simulink model "INS"  (R2018b)
settings: configuration reference "ins_config" (kept outside this file)
values from neighbouring files (symbols this model uses):
  INS_EXPORT = Simulink.Parameter(INS_EXPORT_VALUE)    [ins_model_init.m]
  INS_PARAM = Simulink.Parameter(INS_PARAM_VALUE)    [ins_model_init.m]
undefined symbols (not defined in the file or in its folder): DiscIntNeverNeededParam, INS_CONST, INS_EXPORT_VALUE, Sensor_Meas
libraries: simulink x131, FMT_Model_Lib x48
(part 4 of 6)

== system INS/Data_Fusion/Translation_Filter/TF_Data_PreProcess/Sensor_Process/TF_Sensor_Status/ExternalPos_Status ==
  Sensor_Data : Inport
  Bus Creator : BusCreator  Inputs=2
  Bus Selector : BusSelector  OutputSignals=ExternalPos_Data.pos_valid,ExternalPos_Data.height_valid
  Signal Copy : SignalConversion  OverrideOpt=off
  Signal Copy1 : SignalConversion  OverrideOpt=off
  ExtPos_Status : Outport
  wires:
  Signal Copy/1 -> Bus Creator/1  "pos_valid"
  Sensor_Data/1 -> Bus Selector/1
  Bus Creator/1 -> ExtPos_Status/1
  Bus Selector/1 -> Signal Copy/1  "<pos_valid>"
  Bus Selector/2 -> Signal Copy1/1  "<height_valid>"
  Signal Copy1/1 -> Bus Creator/2  "height_valid"

== system INS/Data_Fusion/Translation_Filter/TF_Data_PreProcess/Sensor_Process/TF_Sensor_Status/GPS_Status ==
  Sensor_Data : Inport
  Rotation_Data : Inport  Port=2
  Bus Creator : BusCreator  Inputs=6
  Bus Selector : BusSelector  OutputSignals=GPS_Data.GPS_valid,GPS_Data.spd_quality,GPS_Data.pos_quality,GPS_Data.alt_quality,GPS_Data.fixType
  Bus Selector1 : BusSelector  OutputSignals=standstill
  Compare To Constant : simulink/Logic and Bit Operations/Compare To Constant  relop===  const=6  OutDataTypeStr=boolean
  Relay : Relay  OnSwitchValue=0.7  OffSwitchValue=0.4
  Relay1 : Relay  OnSwitchValue=0.7  OffSwitchValue=0.5
  Relay2 : Relay  OnSwitchValue=0.7  OffSwitchValue=0.6
  Signal Copy : SignalConversion  OverrideOpt=off
  Signal Copy1 : SignalConversion  OverrideOpt=off
  GPS_Status : Outport
  wires:
  Bus Creator/1 -> GPS_Status/1
  Relay1/1 -> Bus Creator/3  "pos_valid"
  Relay/1 -> Bus Creator/2  "spd_valid"
  Signal Copy/1 -> Bus Creator/1  "gps_vaid"
  Bus Selector/3 -> Relay1/1  "<pos_quality>"
  Bus Selector/2 -> Relay/1  "<spd_quality>"
  Bus Selector/1 -> Signal Copy/1  "<GPS_valid>"
  Sensor_Data/1 -> Bus Selector/1
  Bus Selector/4 -> Relay2/1  "<alt_quality>"
  Relay2/1 -> Bus Creator/4  "alt_valid"
  Bus Selector/5 -> Compare To Constant/1  "<fixType>"
  Compare To Constant/1 -> Bus Creator/5  "rtk_valid"
  Rotation_Data/1 -> Bus Selector1/1
  Bus Selector1/1 -> Signal Copy1/1  "<standstill>"
  Signal Copy1/1 -> Bus Creator/6  "standstill"

== system INS/Data_Fusion/Translation_Filter/TF_Data_PreProcess/Sensor_Process/TF_Sensor_Status/OpticalFlow_Status ==
  Sensor_Data : Inport
  Bus Creator : BusCreator  Inputs=1
  Bus Selector : BusSelector  OutputSignals=OpticalFlow_Data.valid
  Signal Copy : SignalConversion  OverrideOpt=off
  OptFlow_Status : Outport
  wires:
  Signal Copy/1 -> Bus Creator/1  "optflow_valid"
  Sensor_Data/1 -> Bus Selector/1
  Bus Creator/1 -> OptFlow_Status/1
  Bus Selector/1 -> Signal Copy/1  "<valid>"

== system INS/Data_Fusion/Translation_Filter/TF_Data_PreProcess/Sensor_Process/TF_Sensor_Status/Rangefinder_Status ==
  Sensor_Data : Inport
  Bus Creator : BusCreator  Inputs=1
  Bus Selector : BusSelector  OutputSignals=Rangefinder_Data.valid
  Signal Copy : SignalConversion  OverrideOpt=off
  Rf_Status : Outport
  wires:
  Bus Selector/1 -> Signal Copy/1  "<valid>"
  Bus Creator/1 -> Rf_Status/1
  Sensor_Data/1 -> Bus Selector/1
  Signal Copy/1 -> Bus Creator/1  "rf_valid"

== system INS/Data_Fusion/Translation_Filter/TF_Data_PreProcess/TF_Data_Post_Process/GPS_OFFSET_Compensation/GPS_POS_Compensation ==
  Rotation_Data : Inport
  TF_Data : Inport  Port=2
  GPS_Offset : Inport  Port=3
  Bus Selector1 : BusSelector  OutputSignals=M_OB
  Multiply2 : Product  Multiplication=Matrix(*)
  Reshape : Reshape  OutputDimensionality=Column vector (2-D)
  Sum1 : Sum  Inputs=|-+
  WGS_To_Global : Subsystem
  pos_O_m : Outport
  wires:
  WGS_To_Global/1(pos_O_m) -> Reshape/1
  TF_Data/1 -> WGS_To_Global/1(TF_Data)
  GPS_Offset/1 -> Multiply2/2
  Rotation_Data/1 -> Bus Selector1/1
  Bus Selector1/1 -> Multiply2/1  "<M_OB>"
  Reshape/1 -> Sum1/2
  Multiply2/1 -> Sum1/1
  Sum1/1 -> pos_O_m/1

== system INS/Data_Fusion/Translation_Filter/TF_Data_PreProcess/TF_Data_Post_Process/GPS_OFFSET_Compensation/GPS_VEL_Compensation ==
  Rotation_Data : Inport
  TF_Data : Inport  Port=2
  GPS_Offset : Inport  Port=3
  Bus Selector2 : BusSelector  OutputSignals=M_OB
  Bus Selector3 : BusSelector  OutputSignals=Sensor_Meas.GPS_Meas.vn_mPs,Sensor_Meas.GPS_Meas.ve_mPs,Sensor_Meas.GPS_Meas.vd_mPs
  Bus Selector4 : BusSelector  OutputSignals=gyr_B_radPs
  Cross Product : FMT_Model_Lib/Math/Cross Product
      settings: SourceProductName=FMT Toolbox
  Multiply4 : Product  Multiplication=Matrix(*)
  Mux1 : Mux  Inputs=3
  Reshape : Reshape  OutputDimensionality=Column vector (2-D)
  Sum : Sum  Inputs=+-|
  delay : Subsystem
  vel_O_mPs : Outport
  wires:
  Bus Selector3/3 -> Mux1/3  "<vd_mPs>"
  Bus Selector3/2 -> Mux1/2  "<ve_mPs>"
  Mux1/1 -> Reshape/1
  TF_Data/1 -> Bus Selector3/1
  Rotation_Data/1 -> Bus Selector2/1, Bus Selector4/1
  Bus Selector4/1 -> Cross Product/1  "<gyr_B_radPs>"
  Bus Selector3/1 -> Mux1/1  "<vn_mPs>"
  GPS_Offset/1 -> Cross Product/2
  Reshape/1 -> Sum/1
  Bus Selector2/1 -> Multiply4/1  "<M_OB>"
  Multiply4/1 -> Sum/2
  Cross Product/1 -> delay/1(u)  "gps_vel_offset"
  delay/1(y) -> Multiply4/2
  Sum/1 -> vel_O_mPs/1

== system INS/Data_Fusion/Translation_Filter/TF_Data_PreProcess/Transfer_Filter_Control/Sensor_Valid/Horizon_Sensor_Valid ==
  Sensor_Enable : Inport
  Bus Selector1 : BusSelector  OutputSignals=horizon_select.gps_enable,horizon_select.optflow_enable,horizon_select.extpos_enable,horizon_select.airspeed_enable
  Logical Operator : Logic  Operator=OR  Inputs=3  AllPortsSameDT=off  OutDataTypeStr=boolean
  valid_hold : Subsystem  mask{time_out=1000}
      mask prompts: time_out "timeout in ms"
  valid_hold1 : Subsystem  mask{time_out=1000}
      mask prompts: time_out "timeout in ms"
  valid_hold2 : Subsystem  mask{time_out=1000}
      mask prompts: time_out "timeout in ms"
  lon_lat_valid : Outport
  xy_R_valid : Outport  Port=2
  airspeed_valid : Outport  Port=3
  wires:
  Sensor_Enable/1 -> Bus Selector1/1
  Bus Selector1/1 -> Logical Operator/1, valid_hold/1(u)  "<gps_enable>"
  valid_hold/1(y) -> lon_lat_valid/1
  valid_hold1/1(y) -> xy_R_valid/1
  Bus Selector1/2 -> Logical Operator/2  "<optflow_enable>"
  Logical Operator/1 -> valid_hold1/1(u)
  Bus Selector1/3 -> Logical Operator/3  "<extpos_enable>"
  valid_hold2/1(y) -> airspeed_valid/1
  Bus Selector1/4 -> valid_hold2/1(u)  "<airspeed_enable>"

== system INS/Data_Fusion/Translation_Filter/TF_Data_PreProcess/Transfer_Filter_Control/Sensor_Valid/Vertical_Sensor_Valid ==
  Sensor_Enable : Inport
  Bus Selector1 : BusSelector  OutputSignals=vert_select.gps_enable,vert_select.baro_enable,vert_select.extpos_enable,vert_select.rf_enable
  Logical Operator : Logic  Operator=OR  Inputs=4  AllPortsSameDT=off  OutDataTypeStr=boolean
  valid_hold : Subsystem  mask{time_out=1000}
      mask prompts: time_out "timeout in ms"
  valid_hold1 : Subsystem  mask{time_out=1000}
      mask prompts: time_out "timeout in ms"
  valid_hold2 : Subsystem  mask{time_out=1000}
      mask prompts: time_out "timeout in ms"
  altitude_valid : Outport
  h_R_valid : Outport  Port=2
  h_AGL_valid : Outport  Port=3
  wires:
  Sensor_Enable/1 -> Bus Selector1/1
  Bus Selector1/1 -> Logical Operator/1, valid_hold/1(u)  "<gps_enable>"
  Bus Selector1/2 -> Logical Operator/2  "<baro_enable>"
  Logical Operator/1 -> valid_hold1/1(u)
  valid_hold/1(y) -> altitude_valid/1
  valid_hold1/1(y) -> h_R_valid/1
  Bus Selector1/4 -> Logical Operator/4, valid_hold2/1(u)  "<rf_enable>"
  valid_hold2/1(y) -> h_AGL_valid/1
  Bus Selector1/3 -> Logical Operator/3  "<extpos_enable>"

== system INS/Data_Fusion/Translation_Filter/TF_Data_PreProcess/Transfer_Filter_Control/WGS84_Reference/Bus_Constructor ==
  WGS84_pos_ref : Inport
  WGS84_dpos_ref : Inport  Port=2
  WGS84_hgt_ref : Inport  Port=3
  WGS84_dhgt_ref : Inport  Port=4
  Bus Creator : BusCreator  Inputs=2
  Bus Creator1 : BusCreator  Inputs=3
  Bus Creator2 : BusCreator  Inputs=3
  Demux : Demux  Outputs=2
  Demux1 : Demux  Outputs=2
  WGS84_Ref : Outport
  wires:
  Bus Creator/1 -> WGS84_Ref/1
  Demux/1 -> Bus Creator1/1  "dx_dlat_0"
  Demux1/1 -> Bus Creator2/1  "lat_0_rad"
  Demux/2 -> Bus Creator1/2  "dy_dlon_0"
  Demux1/2 -> Bus Creator2/2  "lon_0_rad"
  Bus Creator2/1 -> Bus Creator/2  "WGS84_pos_ref"
  WGS84_dhgt_ref/1 -> Bus Creator1/3  "dz_dh_0"
  WGS84_hgt_ref/1 -> Bus Creator2/3  "h_0_m"
  Bus Creator1/1 -> Bus Creator/1  "WGS84_derivatives_ref"
  WGS84_dpos_ref/1 -> Demux/1
  WGS84_pos_ref/1 -> Demux1/1

== system INS/Data_Fusion/Translation_Filter/TF_Data_PreProcess/Transfer_Filter_Control/WGS84_Reference/Bus_Select ==
  Sensor_Meas : Inport
  Bus Selector1 : BusSelector  OutputSignals=GPS_Meas.dx_dlat,GPS_Meas.dy_dlon,GPS_Meas.dz_dh,GPS_Meas.lat_rad,GPS_Meas.lon_rad,GPS_Meas.h_m
  Mux : Mux  Inputs=3
  Mux1 : Mux  Inputs=3
  WGS84_derivatives : Outport
  WGS84_position : Outport  Port=2
  wires:
  Mux1/1 -> WGS84_position/1
  Sensor_Meas/1 -> Bus Selector1/1
  Mux/1 -> WGS84_derivatives/1
  Bus Selector1/6 -> Mux1/3  "<h_m>"
  Bus Selector1/5 -> Mux1/2  "<lon_rad>"
  Bus Selector1/4 -> Mux1/1  "<lat_rad>"
  Bus Selector1/3 -> Mux/3  "<dz_dh>"
  Bus Selector1/2 -> Mux/2  "<dy_dlon>"
  Bus Selector1/1 -> Mux/1  "<dx_dlat>"

== system INS/Data_Fusion/Translation_Filter/TF_Data_PreProcess/Transfer_Filter_Control/WGS84_Reference/Height_Ref ==
  Translation_Data : Inport
  Sensor_Valid : Inport  Port=2
  WGS84_derivatives : Inport  Port=3
  WGS84_position : Inport  Port=4
  Bus Selector1 : BusSelector  OutputSignals=h_R_m
  Bus Selector2 : BusSelector  OutputSignals=altitude_valid
  Delay : Delay  DelayLength=1
  Delay1 : Delay  DelayLength=1
  Detect Rise Positive3 : simulink/Logic and Bit Operations/Detect Rise Positive  vinit=0  OutDataTypeStr=boolean
  Selector : Selector  InputPortWidth=3  IndexOptions=Index vector (dialog)  Indices=3  OutputSizes=1
  Selector1 : Selector  InputPortWidth=3  IndexOptions=Index vector (dialog)  Indices=3  OutputSizes=1
  Sum : Sum  Inputs=|+-
  Switch1 : Switch  Criteria=u2 > Threshold
  Switch4 : Switch  Criteria=u2 > Threshold
  WGS84_hgt_ref : Outport
  WGS84_dhgt_ref : Outport  Port=2
  wires:
  Delay1/1 -> Switch4/3
  Switch4/1 -> WGS84_hgt_ref/1, Delay1/1
  Detect Rise Positive3/1 -> Switch1/2, Switch4/2
  Bus Selector2/1 -> Detect Rise Positive3/1  "<altitude_valid>"
  WGS84_derivatives/1 -> Selector/1
  Switch1/1 -> WGS84_dhgt_ref/1, Delay/1
  Delay/1 -> Switch1/3
  Sensor_Valid/1 -> Bus Selector2/1
  Translation_Data/1 -> Bus Selector1/1
  Sum/1 -> Switch4/1
  WGS84_position/1 -> Selector1/1
  Selector/1 -> Switch1/1
  Selector1/1 -> Sum/1
  Bus Selector1/1 -> Sum/2  "<h_R_m>"

== system INS/Data_Fusion/Translation_Filter/TF_Data_PreProcess/Transfer_Filter_Control/WGS84_Reference/Position_Ref ==
  Translation_Data : Inport
  Sensor_Valid : Inport  Port=2
  WGS84_derivatives : Inport  Port=3
  WGS84_position : Inport  Port=4
  Bus Selector1 : BusSelector  OutputSignals=x_R_m,y_R_m
  Bus Selector2 : BusSelector  OutputSignals=lon_lat_valid
  Delay : Delay  DelayLength=1
  Delay1 : Delay  DelayLength=1
  Detect Rise Positive3 : simulink/Logic and Bit Operations/Detect Rise Positive  vinit=0  OutDataTypeStr=boolean
  Divide : Product  Inputs=*/
  Mux : Mux  Inputs=2
  Selector : Selector  InputPortWidth=3  IndexOptions=Index vector (dialog)  Indices=[1 2]  OutputSizes=1
  Selector1 : Selector  InputPortWidth=3  IndexOptions=Index vector (dialog)  Indices=[1 2]  OutputSizes=1
  Sum : Sum  Inputs=|+-
  Switch1 : Switch  Criteria=u2 > Threshold
  Switch4 : Switch  Criteria=u2 > Threshold
  WGS84_pos_ref : Outport
  WGS84_dpos_ref : Outport  Port=2
  wires:
  Delay/1 -> Switch4/3
  Bus Selector1/1 -> Mux/1  "<x_R_m>"
  Switch4/1 -> WGS84_pos_ref/1, Delay/1
  Mux/1 -> Divide/1  "dxdy"
  Detect Rise Positive3/1 -> Switch1/2, Switch4/2
  Bus Selector2/1 -> Detect Rise Positive3/1  "<lon_lat_valid>"
  WGS84_derivatives/1 -> Selector/1
  Switch1/1 -> Delay1/1, WGS84_dpos_ref/1
  Delay1/1 -> Switch1/3
  Sensor_Valid/1 -> Bus Selector2/1
  Translation_Data/1 -> Bus Selector1/1
  Sum/1 -> Switch4/1
  Bus Selector1/2 -> Mux/2  "<y_R_m>"
  Divide/1 -> Sum/2  "dlat_dlon"
  WGS84_position/1 -> Selector1/1
  Selector/1 -> Switch1/1, Divide/2  "dxdy_dlatdlon"
  Selector1/1 -> Sum/1

== system INS/Sensor_PreProcess/MAG_PreProcess/Mag_Data_Process/Mag_Quality_Estimate/Mag_Quality/Inclination_Quality_Estimate ==
  nominal_inc_deg : Inport
  mag_normalized_O : Inport  Port=2
  Abs1 : Abs
  Constant2 : Constant  OutDataTypeStr=Inherit: Inherit via back propagation
  Gain1 : Gain  Gain=pi/180
  Saturation : Saturate  UpperLimit=1  LowerLimit=0
  Selector : Selector  InputPortWidth=3  IndexOptions=Index vector (dialog)  Indices=[1 2]  OutputSizes=1
  Selector1 : Selector  InputPortWidth=3  IndexOptions=Index vector (dialog)  Indices=3  OutputSizes=1
  Subtract : Sum  Inputs=+-
  Sum3 : Sum  Inputs=+-|
  Trigonometric Function : Trigonometry  Operator=atan2
  Vector Modulus : FMT_Model_Lib/Math/Vector Modulus
      settings: SourceProductName=FMT Toolbox
  gain : Gain  Gain=2
  inclination_quality : Outport
  wires:
  mag_normalized_O/1 -> Selector1/1, Selector/1
  Trigonometric Function/1 -> Subtract/2
  Vector Modulus/1 -> Trigonometric Function/2
  Abs1/1 -> gain/1
  gain/1 -> Sum3/2
  Gain1/1 -> Subtract/1
  Subtract/1 -> Abs1/1
  Constant2/1 -> Sum3/1
  nominal_inc_deg/1 -> Gain1/1
  Sum3/1 -> Saturation/1
  Selector/1 -> Vector Modulus/1
  Selector1/1 -> Trigonometric Function/1
  Saturation/1 -> inclination_quality/1

== system INS/Sensor_PreProcess/MAG_PreProcess/Mag_Data_Process/Mag_Quality_Estimate/Mag_Quality/Intensity_Quality_Estimate ==
  mag_normalized_O : Inport
  Abs : Abs
  Constant1 : Constant  OutDataTypeStr=Inherit: Inherit via back propagation
  Nominal_Magnitude : Constant  OutDataTypeStr=Inherit: Inherit via back propagation
  Saturation : Saturate  UpperLimit=1  LowerLimit=0
  Subtract : Sum  Inputs=+-
  Sum : Sum  Inputs=+-|
  Vector Modulus : FMT_Model_Lib/Math/Vector Modulus
      settings: SourceProductName=FMT Toolbox
  gain : Gain
  intensity_quality : Outport
  wires:
  Constant1/1 -> Sum/1
  Vector Modulus/1 -> Subtract/2
  Subtract/1 -> Abs/1
  Sum/1 -> Saturation/1
  Nominal_Magnitude/1 -> Subtract/1
  Saturation/1 -> intensity_quality/1
  Abs/1 -> gain/1  "magnitude_error"
  gain/1 -> Sum/2
  mag_normalized_O/1 -> Vector Modulus/1

== system INS/Data_Fusion/Rotation_Filter/AHRS/Correct/Attitude_Correction/Attitude_Correct/Acc_Correct ==
  acc_meas_valid : Inport
  acc_meas_O_mPs2 : Inport  Port=2
  acc_est_O_mPs2 : Inport  Port=3
  Heading_Correct : Subsystem
  Sum : Sum  Inputs=|++
  Verticle_Correct : Subsystem
  att_correct : Outport
  wires:
  acc_meas_valid/1 -> Heading_Correct/3(acc_meas_valid)
  Verticle_Correct/1(vert_correct) -> Sum/1  "vert_correct"
  Heading_Correct/1(heading_correct) -> Sum/2  "heading_correct"
  acc_meas_O_mPs2/1 -> Verticle_Correct/2(acc_meas_O_mPs2), Heading_Correct/2(acc_meas_O_mPs2)
  acc_est_O_mPs2/1 -> Verticle_Correct/1(acc_est_O_mPs2), Heading_Correct/1(acc_est_O_mPs2)
  Sum/1 -> att_correct/1

== system INS/Data_Fusion/Rotation_Filter/AHRS/Correct/Attitude_Correction/Attitude_Correct/Acc_Estimator ==
  RF_Data : Inport
  Sensor_Data : Inport  Port=2
  Rotation_Data : Inport  Port=3
  Estimate_Acc : Subsystem
  Measure_Acc : Subsystem
  Multiply : Product  OutDataTypeStr=single
  Sum2 : Sum  Inputs=++|
  gravity : Constant  Value=[0;0;-INS_CONST.g]  VectorParams1D=off  OutDataTypeStr=single
  acc_meas_valid : Outport
  acc_meas_O_mPs2 : Outport  Port=2
  acc_est_O_mPs2 : Outport  Port=3
  wires:
  Measure_Acc/1(gps_meas_valid) -> Estimate_Acc/1(gps_meas_valid), acc_meas_valid/1, Multiply/1
  Sum2/1 -> acc_meas_O_mPs2/1
  Sensor_Data/1 -> Estimate_Acc/2(Sensor_Data), Measure_Acc/2(Sensor_Data)
  gravity/1 -> Sum2/1
  Multiply/1 -> Sum2/2
  Measure_Acc/2(gps_meas_acc) -> Multiply/2
  Rotation_Data/1 -> Estimate_Acc/3(Rotation_Data)
  Estimate_Acc/1(acc_est_O_mPs2) -> acc_est_O_mPs2/1
  RF_Data/1 -> Measure_Acc/1(RF_Data)

== system INS/Data_Fusion/Rotation_Filter/AHRS/Correct/Attitude_Correction/ExternalPsi_Correct/Bias_Estimation ==
  bias_update : Inport
  psi_meas : Inport  Port=2
  psi_est : Inport  Port=3
  Bias : Subsystem
  Constant : Constant  Value=INS_PARAM.EXT_PSI_BIAS_EST_EN
  Delay : Delay  DelayLength=1
  Multiply : Product
  Switch : Switch  Criteria=u2 > Threshold  OutDataTypeStr=single
  bias : Outport
  wires:
  Delay/1 -> Switch/3
  Bias/1(bias) -> Switch/1
  Multiply/1 -> Delay/1, bias/1
  psi_meas/1 -> Bias/2(psi_meas)
  psi_est/1 -> Bias/1(psi_est)
  bias_update/1 -> Switch/2  "ext_psi_bias_update"
  Switch/1 -> Multiply/2
  Constant/1 -> Multiply/1

== system INS/Data_Fusion/Rotation_Filter/AHRS/Correct/Attitude_Correction/ExternalPsi_Correct/psi_err_saturation ==
  psi_err_in : Inport
  Abs : Abs
  Compare To Constant : simulink/Logic and Bit Operations/Compare To Constant  relop=>  const=pi  OutDataTypeStr=boolean
  Constant : Constant  Value=2*pi  OutDataTypeStr=single
  Multiply : Product
  Sign : Signum
  Subtract : Sum  Inputs=-+
  Switch : Switch  Criteria=u2 > Threshold
  psi_err_rad : Outport
  wires:
  Multiply/1 -> Switch/1
  Sign/1 -> Multiply/2
  Subtract/1 -> Multiply/1
  Constant/1 -> Subtract/1
  Switch/1 -> psi_err_rad/1
  Compare To Constant/1 -> Switch/2
  Abs/1 -> Compare To Constant/1, Subtract/2
  psi_err_in/1 -> Abs/1, Switch/3, Sign/1

== system INS/Data_Fusion/Rotation_Filter/AHRS/Correct/Attitude_Correction/GPS_Heading_Correct/psi_err_saturation ==
  psi_err_in : Inport
  Abs : Abs
  Compare To Constant : simulink/Logic and Bit Operations/Compare To Constant  relop=>  const=pi  OutDataTypeStr=boolean
  Constant : Constant  Value=2*pi  OutDataTypeStr=single
  Multiply : Product
  Sign : Signum
  Subtract : Sum  Inputs=-+
  Switch : Switch  Criteria=u2 > Threshold
  psi_err_rad : Outport
  wires:
  Multiply/1 -> Switch/1
  Sign/1 -> Multiply/2
  Subtract/1 -> Multiply/1
  Constant/1 -> Subtract/1
  Switch/1 -> psi_err_rad/1
  Compare To Constant/1 -> Switch/2
  Abs/1 -> Compare To Constant/1, Subtract/2
  psi_err_in/1 -> Abs/1, Switch/3, Sign/1

== system INS/Data_Fusion/Rotation_Filter/AHRS/Correct/Attitude_Correction/Mag_Correct/Mag_Control ==
  RF_Data : Inport
  Rotation_Data : Inport  Port=2
  Sensor_Data : Inport  Port=3
  Translation_Data : Inport  Port=4
  Bus Selector3 : BusSelector  OutputSignals=mag_enable
  Detect Increase1 : simulink/Logic and Bit Operations/Detect Increase  vinit=0.0  OutDataTypeStr=boolean
  Hover : Subsystem
  Hover_Mag_Correcrt : Subsystem
  Logical Operator4 : Logic  Operator=OR  AllPortsSameDT=off  OutDataTypeStr=boolean
  use_mag : Outport
  mag_bias_update : Outport  Port=2
  wires:
  Rotation_Data/1 -> Hover/1(Rotation_Data)
  Detect Increase1/1 -> mag_bias_update/1  "mag_bias_update"
  RF_Data/1 -> Hover_Mag_Correcrt/1(RF_Data), Bus Selector3/1
  Bus Selector3/1 -> Logical Operator4/1  "<mag_enable>"
  Logical Operator4/1 -> Detect Increase1/1, use_mag/1  "use_mag"
  Translation_Data/1 -> Hover/2(Translation_Data)
  Sensor_Data/1 -> Hover_Mag_Correcrt/2(Sensor_Data)
  Hover/1(hover) -> Hover_Mag_Correcrt/3(hover)  "hover"
  Hover_Mag_Correcrt/1(use_mag_when_hover) -> Logical Operator4/2

== system INS/Data_Fusion/Rotation_Filter/AHRS/Correct/Attitude_Correction/Mag_Correct/Mag_Measure ==
  bias_update : Inport
  mag_norm_B : Inport  Port=2
  Rotation_Data : Inport  Port=3
  Bias_Estimation : Subsystem
  Bus Selector : BusSelector  OutputSignals=psi_rad,standstill
  Mag_Heading : Subsystem
  Sum : Sum  Inputs=++|
  psi_meas : Outport
  wires:
  Mag_Heading/1(mag_psi) -> Sum/1, Bias_Estimation/2(psi_meas)
  Rotation_Data/1 -> Mag_Heading/2(Rotation_Data), Bus Selector/1
  mag_norm_B/1 -> Mag_Heading/1(mag_B)
  Bus Selector/1 -> Bias_Estimation/3(psi_est)  "<psi_rad>"
  Sum/1 -> psi_meas/1
  Bias_Estimation/1(bias) -> Sum/2  "psi_bias"
  bias_update/1 -> Bias_Estimation/1(bias_update)
  Bus Selector/2 -> Bias_Estimation/4(standstill)  "<standstill>"

== system INS/Data_Fusion/Rotation_Filter/AHRS/Correct/Attitude_Correction/Mag_Correct/psi_err_saturation ==
  psi_err_in : Inport
  Abs : Abs
  Compare To Constant : simulink/Logic and Bit Operations/Compare To Constant  relop=>  const=pi  OutDataTypeStr=boolean
  Constant : Constant  Value=2*pi  OutDataTypeStr=single
  Multiply : Product
  Sign : Signum
  Subtract : Sum  Inputs=-+
  Switch : Switch  Criteria=u2 > Threshold
  psi_err_rad : Outport
  wires:
  Multiply/1 -> Switch/1
  Sign/1 -> Multiply/2
  Subtract/1 -> Multiply/1
  Constant/1 -> Subtract/1
  Switch/1 -> psi_err_rad/1
  Compare To Constant/1 -> Switch/2
  Abs/1 -> Compare To Constant/1, Subtract/2
  psi_err_in/1 -> Abs/1, Switch/3, Sign/1

== system INS/Data_Fusion/Translation_Filter/CF/Bus_Constructor/Bus_Select/WGS84_Position/WGS84_Position ==
  xyh_R_m : Inport
  TF_Data : Inport  Port=2
  Bus Selector : BusSelector  OutputSignals=TF_Control.WGS84_Ref.WGS84_derivatives_ref.dx_dlat_0,TF_Control.WGS84_Ref.WGS84_derivatives_ref.dy_dlon_0
  Bus Selector1 : BusSelector  OutputSignals=TF_Control.WGS84_Ref.WGS84_pos_ref.lat_0_rad,TF_Control.WGS84_Ref.WGS84_pos_ref.lon_0_rad,TF_Control.WGS84_Ref.WGS84_pos_ref.h_0_m
  Data Type Conversion : DataTypeConversion  OutDataTypeStr=double
  Data Type Conversion1 : DataTypeConversion  OutDataTypeStr=double
  Mux : Mux  Inputs=2
  Mux1 : Mux  Inputs=2
  Mux2 : Mux  Inputs=3
  Selector : Selector  InputPortWidth=3  IndexOptions=Index vector (dialog)  Indices=[1 2]  OutputSizes=1
  Selector1 : Selector  InputPortWidth=3  IndexOptions=Index vector (dialog)  Indices=[3]  OutputSizes=1
  Sum : Sum  Inputs=|++
  safe_divide : Subsystem
  WGS84_pos : Outport
  wires:
  Selector/1 -> Data Type Conversion/1
  Mux/1 -> safe_divide/2(u2)
  Selector1/1 -> Data Type Conversion1/1
  Data Type Conversion1/1 -> Mux1/2
  Bus Selector/1 -> Mux/1  "<dx_dlat_0>"
  xyh_R_m/1 -> Selector1/1, Selector/1
  Bus Selector/2 -> Mux/2  "<dy_dlon_0>"
  safe_divide/1(y) -> Mux1/1
  Data Type Conversion/1 -> safe_divide/1(u1)
  Mux1/1 -> Sum/1
  Bus Selector1/2 -> Mux2/2  "<lon_0_rad>"
  TF_Data/1 -> Bus Selector1/1, Bus Selector/1
  Bus Selector1/3 -> Mux2/3  "<h_0_m>"
  Bus Selector1/1 -> Mux2/1  "<lat_0_rad>"
  Mux2/1 -> Sum/2
  Sum/1 -> WGS84_pos/1

== system INS/Data_Fusion/Translation_Filter/CF/Horizontal_Filter/Correct/Airspeed Correct/Airspeed_Correct ==
  TF_Data : Inport
  X_Predict : Inport  Port=2
  Enable : EnablePort  StatesWhenEnabling=reset
  Bus Selector : BusSelector  OutputSignals=TF_Control.sensor_valid.airspeed_valid
  Bus Selector1 : BusSelector  OutputSignals=Sensor_Meas.Airspeed_Meas.timestamp_ms
  Detect Change : simulink/Logic and Bit Operations/Detect Change  vinit=0  OutDataTypeStr=boolean
  Detect Increase : simulink/Logic and Bit Operations/Detect Increase  vinit=0.0  OutDataTypeStr=boolean
  Error_Integrate : Subsystem
  Error_Scaling : Subsystem
  Estimate_State : Subsystem
  Measurement : Subsystem
  Sum : Sum  Inputs=|-+
  Sum1 : Sum  Inputs=++|
  X_Next : Outport
  wires:
  Error_Scaling/1(err_out) -> Error_Integrate/1(error)
  Detect Change/1 -> Error_Integrate/2(update)
  Bus Selector/1 -> Detect Increase/1  "<airspeed_valid>"
  X_Predict/1 -> Sum1/1, Estimate_State/1(X)
  Sum1/1 -> X_Next/1
  Error_Integrate/1(corr) -> Sum1/2
  Bus Selector1/1 -> Detect Change/1  "<timestamp_ms>"
  Sum/1 -> Error_Scaling/1(err_in)  "airspeed_error_hor_O"
  TF_Data/1 -> Bus Selector1/1, Bus Selector/1, Measurement/1(TF_Data)
  Measurement/1(Z) -> Sum/2  "airspeed_meas_hor_O"
  Estimate_State/1(HX) -> Sum/1  "airspeed_state_hor_O"
  Detect Increase/1 -> Estimate_State/2(reset)

== system INS/Data_Fusion/Translation_Filter/CF/Horizontal_Filter/Correct/ExternalPos Correct/ExternalPos_Correct ==
  TF_Data : Inport
  X_Predict : Inport  Port=2
  Enable : EnablePort  StatesWhenEnabling=reset
  Bus Selector : BusSelector  OutputSignals=TF_Control.pos_reset
  Bus Selector1 : BusSelector  OutputSignals=Sensor_Meas.ExtPos_Meas.timestamp_ms
  Detect Change : simulink/Logic and Bit Operations/Detect Change  vinit=0  OutDataTypeStr=boolean
  Error_Integrate : Subsystem
  Error_Scaling : Subsystem
  Estimate_State : Subsystem
  Logical Operator : Logic  Operator=OR  AllPortsSameDT=off  OutDataTypeStr=boolean
  Measurement : Subsystem
  Sum : Sum  Inputs=|-+
  Sum1 : Sum  Inputs=++|
  X_Next : Outport
  wires:
  Estimate_State/1(HX) -> Sum/1  "extpos_state_hor_O"
  Measurement/1(Z) -> Sum/2  "extpos_meas_hor_O"
  TF_Data/1 -> Measurement/2(TF_Data), Bus Selector/1, Bus Selector1/1
  Sum/1 -> Error_Scaling/1(err_in)  "extpos_error_hor_O"
  Bus Selector1/1 -> Detect Change/1  "<timestamp_ms>"
  Error_Integrate/1(corr) -> Sum1/2  "corr_1"
  Sum1/1 -> X_Next/1
  X_Predict/1 -> Measurement/1(X), Estimate_State/1(X), Sum1/1
  Bus Selector/1 -> Estimate_State/2(reset)  "<pos_reset>"
  Logical Operator/1 -> Error_Integrate/2(update)
  Detect Change/1 -> Logical Operator/2
  Measurement/2(bias_update) -> Logical Operator/1
  Error_Scaling/1(err_out) -> Error_Integrate/1(error)

== system INS/Data_Fusion/Translation_Filter/CF/Horizontal_Filter/Correct/GPS Correct/GPS_Correct ==
  TF_Data : Inport
  X_Predict : Inport  Port=2
  Enable : EnablePort  StatesWhenEnabling=reset
  Bus Selector : BusSelector  OutputSignals=TF_Control.pos_reset
  Bus Selector1 : BusSelector  OutputSignals=Sensor_Meas.GPS_Meas.timestamp_ms
  Bus Selector2 : BusSelector  OutputSignals=Sensor_Status.GPS_Status.rtk_valid
  Detect Change : simulink/Logic and Bit Operations/Detect Change  vinit=0  OutDataTypeStr=boolean
  Error_Integrate : Subsystem
  Error_Scaling : Subsystem
  Estimate_State : Subsystem
  Logical Operator : Logic  Operator=OR  AllPortsSameDT=off  OutDataTypeStr=boolean
  Measurement : Subsystem
  Sum : Sum  Inputs=|-+
  Sum1 : Sum  Inputs=++|
  X_Next : Outport
  wires:
  Estimate_State/1(HX) -> Sum/1  "gps_state_hor_O"
  Measurement/1(Z) -> Sum/2  "gps_meas_hor_O"
  TF_Data/1 -> Bus Selector2/1, Bus Selector/1, Measurement/2(TF_Data), Bus Selector1/1
  Sum/1 -> Error_Scaling/1(err_in)  "gps_error_hor_O"
  Bus Selector1/1 -> Detect Change/1  "<timestamp_ms>"
  Error_Integrate/1(corr) -> Sum1/2
  Sum1/1 -> X_Next/1
  X_Predict/1 -> Estimate_State/1(X), Measurement/1(X), Sum1/1
  Bus Selector/1 -> Estimate_State/2(reset)  "<pos_reset>"
  Logical Operator/1 -> Error_Integrate/2(update)
  Detect Change/1 -> Logical Operator/2
  Measurement/2(bias_update) -> Logical Operator/1
  Error_Scaling/1(err_out) -> Error_Integrate/1(error)
  Bus Selector2/1 -> Error_Scaling/2(rtk_valid)  "<rtk_valid>"

== system INS/Data_Fusion/Translation_Filter/CF/Horizontal_Filter/Correct/OptFlow Correct/OptFlow_Correct ==
  TF_Data : Inport
  X_Predict : Inport  Port=2
  Enable : EnablePort  StatesWhenEnabling=reset
  Bus Selector : BusSelector  OutputSignals=TF_Control.pos_reset
  Bus Selector1 : BusSelector  OutputSignals=Sensor_Meas.OptFlow_Meas.timestamp_ms
  Detect Change : simulink/Logic and Bit Operations/Detect Change  vinit=0  OutDataTypeStr=boolean
  Error_Integrate : Subsystem
  Error_Scaling : Subsystem
  Estimate_State : Subsystem
  Measurement : Subsystem
  Sum : Sum  Inputs=|-+
  Sum1 : Sum  Inputs=++|
  X_Next : Outport
  wires:
  Estimate_State/1(HX) -> Sum/1  "optflow_state_O"
  Measurement/1(Z) -> Sum/2  "optflow_meas_O"
  TF_Data/1 -> Bus Selector1/1, Bus Selector/1, Measurement/1(TF_Data)
  Sum/1 -> Error_Scaling/1(err_in)  "optflow_error_O"
  Bus Selector1/1 -> Detect Change/1  "<timestamp_ms>"
  Error_Integrate/1(corr) -> Sum1/2
  Sum1/1 -> X_Next/1
  X_Predict/1 -> Estimate_State/1(X), Sum1/1
  Bus Selector/1 -> Estimate_State/2(reset)  "<pos_reset>"
  Detect Change/1 -> Error_Integrate/2(update)
  Error_Scaling/1(err_out) -> Error_Integrate/1(error)

== system INS/Data_Fusion/Translation_Filter/CF/Horizontal_Filter/Predict/Propagate/States_Init ==
  TF_Data : Inport
  Constant : Constant  Value=[0;0]  VectorParams1D=off  OutDataTypeStr=single
  Constant1 : Constant  Value=0  VectorParams1D=off  OutDataTypeStr=single
  Mux : Mux
  Pos_Init : Subsystem
  Vel_Init : Subsystem
  X_0 : Outport
  wires:
  TF_Data/1 -> Pos_Init/1(TF_Data), Vel_Init/1(TF_Data)
  Constant/1 -> Mux/3  "ba_xy_0"
  Mux/1 -> X_0/1
  Vel_Init/1(vel_NE_0) -> Mux/2  "vel_ne_0"
  Pos_Init/1(XY_0) -> Mux/1  "pos_xy_0"
  Constant1/1 -> Mux/4  "TAS"

== system INS/Data_Fusion/Translation_Filter/CF/Verticle_Filter/Correct/Baro_Correct/Baro_Correct ==
  TF_Data : Inport
  X_Predict : Inport  Port=2
  Enable : EnablePort  StatesWhenEnabling=reset
  Bus Selector : BusSelector  OutputSignals=TF_Control.height_reset
  Bus Selector1 : BusSelector  OutputSignals=Sensor_Meas.Baro_Meas.timestamp_ms
  Demux : Demux  Outputs=3
  Detect Change : simulink/Logic and Bit Operations/Detect Change  vinit=0  OutDataTypeStr=boolean
  Error_Hold : Subsystem
  Error_Scaling : Subsystem  mask{w=1.2}
      mask prompts: w "omega"
  Estimate_States : Subsystem
  Logical Operator : Logic  Operator=OR  AllPortsSameDT=off  OutDataTypeStr=boolean
  Measurement : Subsystem
  Mux : Mux  Inputs=3
  Saturation : Saturate
  Sum : Sum  Inputs=|-+
  Sum1 : Sum  Inputs=++|
  X_Next : Outport
  wires:
  Estimate_States/1(HX) -> Sum/1  "baro_state_vert_O"
  Measurement/1(Z) -> Sum/2  "baro_meas_vert_O"
  TF_Data/1 -> Bus Selector/1, Measurement/2(TF_Data), Bus Selector1/1
  Sum/1 -> Error_Scaling/1(errror_in)  "baro_error_vert_O"
  Bus Selector1/1 -> Detect Change/1  "<timestamp_ms>"
  Error_Hold/1(out) -> Sum1/2
  Sum1/1 -> Demux/1
  X_Predict/1 -> Measurement/1(X), Estimate_States/1(X), Sum1/1
  Bus Selector/1 -> Estimate_States/2(reset)  "<height_reset>"
  Logical Operator/1 -> Error_Hold/2(update)
  Detect Change/1 -> Logical Operator/2
  Measurement/2(bias_update) -> Logical Operator/1
  Error_Scaling/1(errror_out) -> Error_Hold/1(in)
  Demux/3 -> Saturation/1
  Mux/1 -> X_Next/1
  Saturation/1 -> Mux/3
  Demux/2 -> Mux/2
  Demux/1 -> Mux/1

== system INS/Data_Fusion/Translation_Filter/CF/Verticle_Filter/Correct/ExternalPos_Correct/ExternalPos_Correct ==
  TF_Data : Inport
  X_Predict : Inport  Port=2
  Enable : EnablePort  StatesWhenEnabling=reset
  Bus Selector : BusSelector  OutputSignals=TF_Control.height_reset
  Bus Selector1 : BusSelector  OutputSignals=Sensor_Meas.ExtPos_Meas.timestamp_ms
  Detect Change : simulink/Logic and Bit Operations/Detect Change  vinit=0  OutDataTypeStr=boolean
  Error_Hold : Subsystem
  Error_Scaling : Subsystem  mask{w=1.2}
      mask prompts: w "omega"
  Estimate_States : Subsystem
  Logical Operator : Logic  Operator=OR  AllPortsSameDT=off  OutDataTypeStr=boolean
  Measurement : Subsystem
  Sum : Sum  Inputs=|-+
  Sum1 : Sum  Inputs=++|
  X_Next : Outport
  wires:
  Estimate_States/1(HX) -> Sum/1  "extpos_state_vert_O"
  Measurement/1(Z) -> Sum/2  "extpos_meas_vert_O"
  TF_Data/1 -> Bus Selector/1, Measurement/2(TF_Data), Bus Selector1/1
  Sum/1 -> Error_Scaling/1(errror_in)  "extpos_error_vert_O"
  Bus Selector1/1 -> Detect Change/1  "<timestamp_ms>"
  Error_Hold/1(out) -> Sum1/2
  X_Predict/1 -> Measurement/1(X), Estimate_States/1(X), Sum1/1
  Bus Selector/1 -> Estimate_States/2(reset)  "<height_reset>"
  Logical Operator/1 -> Error_Hold/2(update)
  Detect Change/1 -> Logical Operator/2
  Measurement/2(bias_update) -> Logical Operator/1
  Error_Scaling/1(errror_out) -> Error_Hold/1(in)
  Sum1/1 -> X_Next/1

== system INS/Data_Fusion/Translation_Filter/CF/Verticle_Filter/Correct/GPS_Correct/GPS_Correct ==
  TF_Data : Inport
  X_Predict : Inport  Port=2
  Enable : EnablePort  StatesWhenEnabling=reset
  Bus Selector : BusSelector  OutputSignals=TF_Control.height_reset
  Bus Selector1 : BusSelector  OutputSignals=Sensor_Meas.GPS_Meas.timestamp_ms
  Bus Selector2 : BusSelector  OutputSignals=Sensor_Status.GPS_Status.rtk_valid
  Detect Change : simulink/Logic and Bit Operations/Detect Change  vinit=0  OutDataTypeStr=boolean
  Error_Hold : Subsystem
  Error_Scaling : Subsystem
  Estimate_State : Subsystem
  Logical Operator : Logic  Operator=OR  AllPortsSameDT=off  OutDataTypeStr=boolean
  Measurement : Subsystem
  Sum : Sum  Inputs=|-+
  Sum1 : Sum  Inputs=++|
  X_Next : Outport
  wires:
  Estimate_State/1(HX) -> Sum/1  "gps_state_vert_O"
  Measurement/1(Z) -> Sum/2  "gps_meas_vert_O"
  TF_Data/1 -> Bus Selector2/1, Bus Selector/1, Measurement/2(TF_Data), Bus Selector1/1
  Sum/1 -> Error_Scaling/1(error_in)  "gps_error_vert_O"
  Bus Selector1/1 -> Detect Change/1  "<timestamp_ms>"
  Error_Hold/1(out) -> Sum1/2
  Sum1/1 -> X_Next/1
  X_Predict/1 -> Measurement/1(X), Estimate_State/1(X), Sum1/1
  Bus Selector/1 -> Estimate_State/2(reset)  "<height_reset>"
  Logical Operator/1 -> Error_Hold/2(update)
  Detect Change/1 -> Logical Operator/2
  Measurement/2(bias_update) -> Logical Operator/1
  Error_Scaling/1(error_out) -> Error_Hold/1(in)
  Bus Selector2/1 -> Error_Scaling/2(rtk_valid)  "<rtk_valid>"

== system INS/Data_Fusion/Translation_Filter/CF/Verticle_Filter/Correct/Rf_Correct/Rangefinder_Correct ==
  TF_Data : Inport
  X_Predict : Inport  Port=2
  Enable : EnablePort  StatesWhenEnabling=reset
  Bus Selector : BusSelector  OutputSignals=TF_Control.height_reset
  Bus Selector1 : BusSelector  OutputSignals=Sensor_Meas.Rf_Meas.timestamp_ms
  Detect Change : simulink/Logic and Bit Operations/Detect Change  vinit=0  OutDataTypeStr=boolean
  Error_Hold : Subsystem
  Error_Scaling : Subsystem
  Estimate_State : Subsystem
  Logical Operator : Logic  Operator=OR  AllPortsSameDT=off  OutDataTypeStr=boolean
  Measurement : Subsystem
  Sum : Sum  Inputs=|-+
  Sum1 : Sum  Inputs=++|
  X_Next : Outport
  rf_bias : Outport  Port=2
  wires:
  Estimate_State/1(HX) -> Sum/1  "rf_state"
  Measurement/1(Z) -> Sum/2  "rf_meas"
  TF_Data/1 -> Bus Selector/1, Measurement/2(TF_Data), Bus Selector1/1
  Sum/1 -> Error_Scaling/1(error_in)  "rf_error"
  Bus Selector1/1 -> Detect Change/1  "<timestamp_ms>"
  Error_Hold/1(out) -> Sum1/2
  Sum1/1 -> X_Next/1
  X_Predict/1 -> Measurement/1(X), Estimate_State/1(X), Sum1/1
  Bus Selector/1 -> Estimate_State/2(reset)  "<height_reset>"
  Logical Operator/1 -> Error_Hold/2(update)
  Detect Change/1 -> Logical Operator/2
  Measurement/2(bias_update) -> Logical Operator/1
  Error_Scaling/1(error_out) -> Error_Hold/1(in)
  Measurement/3(bias) -> rf_bias/1

== system INS/Data_Fusion/Translation_Filter/CF/Verticle_Filter/Predict/Propagate/States_Init ==
  TF_Data : Inport
  Constant : Constant  Value=0  OutDataTypeStr=single
  Height_Init : Subsystem
  Mux : Mux  Inputs=3
  Velocity_Init : Subsystem
  X_0 : Outport
  wires:
  Constant/1 -> Mux/3  "ba_z_0"
  Mux/1 -> X_0/1
  Height_Init/1(h_0) -> Mux/1  "h_0"
  Velocity_Init/1(vel_D) -> Mux/2  "vel_D_0"
  TF_Data/1 -> Velocity_Init/1(TF_Data), Height_Init/1(TF_Data)

== system INS/Data_Fusion/Translation_Filter/TF_Data_PreProcess/Sensor_Process/TF_Sensor_Measures/ExternalPos_Meas/External_Pos_PreProcess ==
  Sensor_Data : Inport
  Rotation_Data : Inport  Port=2
  Bus Selector2 : BusSelector  OutputSignals=ExternalPos_Data.x,ExternalPos_Data.y,ExternalPos_Data.h
  Bus Selector5 : BusSelector  OutputSignals=ExternalPos_Data.timestamp
  Constant2 : Constant  Value=INS_PARAM.EXT_PSI_OFS
  Demux : Demux  Outputs=3
  Multiply : Product  Multiplication=Matrix(*)
  Mux : Mux  Inputs=3
  Psi To DCM : FMT_Model_Lib/Transformation/Psi To DCM
      settings: SourceProductName=FMT Toolbox
  Reshape : Reshape  OutputDimensionality=Column vector (2-D)
  Terminator : Terminator
  Transpose : Math  Operator=transpose  SaturateOnIntegerOverflow=on
  timestamp : Outport
  x : Outport  Port=2
  y : Outport  Port=3
  h : Outport  Port=4
  wires:
  Bus Selector2/2 -> Mux/2  "<y>"
  Mux/1 -> Reshape/1  "xyh_local"
  Multiply/1 -> Demux/1
  Demux/1 -> x/1
  Demux/2 -> y/1
  Bus Selector2/3 -> Mux/3  "<h>"
  Reshape/1 -> Multiply/2
  Bus Selector2/1 -> Mux/1  "<x>"
  Demux/3 -> h/1
  Bus Selector5/1 -> timestamp/1  "<timestamp>"
  Sensor_Data/1 -> Bus Selector2/1, Bus Selector5/1
  Transpose/1 -> Multiply/1
  Psi To DCM/1 -> Transpose/1
  Constant2/1 -> Psi To DCM/1
  Rotation_Data/1 -> Terminator/1

== system INS/Data_Fusion/Translation_Filter/TF_Data_PreProcess/TF_Data_Post_Process/GPS_OFFSET_Compensation/GPS_POS_Compensation/WGS_To_Global ==
  TF_Data : Inport
  Bus Selector : BusSelector  OutputSignals=Sensor_Meas.GPS_Meas.lat_rad,Sensor_Meas.GPS_Meas.lon_rad,Sensor_Meas.GPS_Meas.h_m,TF_Control.WGS84_Ref.WGS84_pos_ref.lat_0_rad,TF_Control.WGS84_Ref.WGS84_pos_ref.lon_0_rad,TF_Control.WGS84_Ref.WGS84_pos_ref.h_0_m,TF_Control.WGS84_Ref.WGS84_derivatives_ref.dx_dlat_0,TF_Control.WGS84_Ref.WGS84_derivatives_ref.dy_dlon_0,TF_Control.WGS84_Ref.WGS84_derivatives_ref.dz_dh_0
  Multiply : Product
  Mux : Mux  Inputs=3
  Mux1 : Mux  Inputs=3
  Mux2 : Mux  Inputs=3
  Sum : Sum  Inputs=|+-
  pos_O_m : Outport
  wires:
  Bus Selector/2 -> Mux/2  "<lon_rad>"
  Bus Selector/6 -> Mux1/3  "<h_0_m>"
  Bus Selector/3 -> Mux/3  "<h_m>"
  Mux1/1 -> Sum/2
  Bus Selector/4 -> Mux1/1  "<lat_0_rad>"
  Sum/1 -> Multiply/1
  Mux2/1 -> Multiply/2
  Bus Selector/1 -> Mux/1  "<lat_rad>"
  Bus Selector/5 -> Mux1/2  "<lon_0_rad>"
  Mux/1 -> Sum/1
  TF_Data/1 -> Bus Selector/1
  Multiply/1 -> pos_O_m/1
  Bus Selector/7 -> Mux2/1  "<dx_dlat_0>"
  Bus Selector/8 -> Mux2/2  "<dy_dlon_0>"
  Bus Selector/9 -> Mux2/3  "<dz_dh_0>"

== system INS/Data_Fusion/Translation_Filter/TF_Data_PreProcess/TF_Data_Post_Process/GPS_OFFSET_Compensation/GPS_VEL_Compensation/delay ==
  u : Inport
  Divide : Product  Inputs=*/
  Mux : Mux  Inputs=3
  Selector : Selector  InputPortWidth=3  IndexOptions=Index vector (dialog)  Indices=1  OutputSizes=1
  Selector1 : Selector  InputPortWidth=3  IndexOptions=Index vector (dialog)  Indices=2  OutputSizes=1
  Selector2 : Selector  InputPortWidth=3  IndexOptions=Index vector (dialog)  Indices=3  OutputSizes=1
  gps_vd_delay : Delay  DelayLengthSource=Input port  DelayLength=INS_PARAM.GPS_VEL_DELAY/INS_EXPORT.period  DelayLengthUpperLimit=500  InitialConditionSource=Input port
      settings: InputPortMap=u0,p1,p4
  gps_ve_delay : Delay  DelayLengthSource=Input port  DelayLength=INS_PARAM.GPS_VEL_DELAY/INS_EXPORT.period  DelayLengthUpperLimit=500  InitialConditionSource=Input port
      settings: InputPortMap=u0,p1,p4
  gps_vnl_delay : Delay  DelayLengthSource=Input port  DelayLength=INS_PARAM.GPS_VEL_DELAY/INS_EXPORT.period  DelayLengthUpperLimit=500  InitialConditionSource=Input port
      settings: InputPortMap=u0,p1,p4
  period : Constant  Value=INS_EXPORT.period
  vel_delay : Constant  Value=INS_PARAM.GPS_VEL_DELAY
  y : Outport
  wires:
  u/1 -> Selector2/1, Selector1/1, Selector/1
  Divide/1 -> gps_vnl_delay/2, gps_vd_delay/2, gps_ve_delay/2
  vel_delay/1 -> Divide/1
  Selector/1 -> gps_vnl_delay/3, gps_vnl_delay/1
  Selector1/1 -> gps_ve_delay/3, gps_ve_delay/1
  Selector2/1 -> gps_vd_delay/3, gps_vd_delay/1
  gps_vnl_delay/1 -> Mux/1
  gps_ve_delay/1 -> Mux/2
  gps_vd_delay/1 -> Mux/3
  Mux/1 -> y/1
  period/1 -> Divide/2

== system INS/Data_Fusion/Translation_Filter/TF_Data_PreProcess/Transfer_Filter_Control/Sensor_Valid/Horizon_Sensor_Valid/valid_hold ==
  u : Inport
  Compare To Constant : simulink/Logic and Bit Operations/Compare To Constant  relop=>=  const=time_out  OutDataTypeStr=boolean
  Compare To Constant1 : simulink/Logic and Bit Operations/Compare To Constant  relop=>  const=0  OutDataTypeStr=boolean
  Compare To Constant2 : simulink/Logic and Bit Operations/Compare To Constant  relop=>  const=0  OutDataTypeStr=boolean
  Constant : Constant  Value=INS_EXPORT.period  OutDataTypeStr=Inherit: Inherit via back propagation
  Delay : Delay  DelayLength=1
  Detect Rise Positive : simulink/Logic and Bit Operations/Detect Rise Positive  vinit=0  OutDataTypeStr=boolean
  Discrete-Time Integrator : DiscreteIntegrator  IntegratorMethod=Accumulation: Forward Euler  gainval=1  ExternalReset=level  SampleTime=-1  LimitOutput=on  UpperSaturationLimit=1e6  LowerSaturationLimit=0  ICPrevOutput=DiscIntNeverNeededParam  ICPrevScaledInput=DiscIntNeverNeededParam
  Logical Operator : Logic  Operator=NOT  AllPortsSameDT=off  OutDataTypeStr=boolean
  Logical Operator1 : Logic  Operator=OR  AllPortsSameDT=off  OutDataTypeStr=boolean
  Multiply : Product
  y : Outport
  wires:
  Multiply/1 -> y/1
  Logical Operator1/1 -> Multiply/2, Delay/1
  Detect Rise Positive/1 -> Logical Operator1/1
  Compare To Constant2/1 -> Detect Rise Positive/1
  u/1 -> Compare To Constant1/1, Compare To Constant2/1
  Compare To Constant1/1 -> Discrete-Time Integrator/2
  Constant/1 -> Discrete-Time Integrator/1
  Compare To Constant/1 -> Logical Operator/1
  Logical Operator/1 -> Multiply/1
  Discrete-Time Integrator/1 -> Compare To Constant/1
  Delay/1 -> Logical Operator1/2

== system INS/Data_Fusion/Translation_Filter/TF_Data_PreProcess/Transfer_Filter_Control/Sensor_Valid/Horizon_Sensor_Valid/valid_hold1 ==
  u : Inport
  Compare To Constant : simulink/Logic and Bit Operations/Compare To Constant  relop=>=  const=time_out  OutDataTypeStr=boolean
  Compare To Constant1 : simulink/Logic and Bit Operations/Compare To Constant  relop=>  const=0  OutDataTypeStr=boolean
  Compare To Constant2 : simulink/Logic and Bit Operations/Compare To Constant  relop=>  const=0  OutDataTypeStr=boolean
  Constant : Constant  Value=INS_EXPORT.period  OutDataTypeStr=Inherit: Inherit via back propagation
  Delay : Delay  DelayLength=1
  Detect Rise Positive : simulink/Logic and Bit Operations/Detect Rise Positive  vinit=0  OutDataTypeStr=boolean
  Discrete-Time Integrator : DiscreteIntegrator  IntegratorMethod=Accumulation: Forward Euler  gainval=1  ExternalReset=level  SampleTime=-1  LimitOutput=on  UpperSaturationLimit=1e6  LowerSaturationLimit=0  ICPrevOutput=DiscIntNeverNeededParam  ICPrevScaledInput=DiscIntNeverNeededParam
  Logical Operator : Logic  Operator=NOT  AllPortsSameDT=off  OutDataTypeStr=boolean
  Logical Operator1 : Logic  Operator=OR  AllPortsSameDT=off  OutDataTypeStr=boolean
  Multiply : Product
  y : Outport
  wires:
  Discrete-Time Integrator/1 -> Compare To Constant/1
  Logical Operator/1 -> Multiply/1
  Compare To Constant/1 -> Logical Operator/1
  Constant/1 -> Discrete-Time Integrator/1
  Compare To Constant1/1 -> Discrete-Time Integrator/2
  u/1 -> Compare To Constant2/1, Compare To Constant1/1
  Compare To Constant2/1 -> Detect Rise Positive/1
  Detect Rise Positive/1 -> Logical Operator1/1
  Logical Operator1/1 -> Delay/1, Multiply/2
  Multiply/1 -> y/1
  Delay/1 -> Logical Operator1/2

== system INS/Data_Fusion/Translation_Filter/TF_Data_PreProcess/Transfer_Filter_Control/Sensor_Valid/Horizon_Sensor_Valid/valid_hold2 ==
  u : Inport
  Compare To Constant : simulink/Logic and Bit Operations/Compare To Constant  relop=>=  const=time_out  OutDataTypeStr=boolean
  Compare To Constant1 : simulink/Logic and Bit Operations/Compare To Constant  relop=>  const=0  OutDataTypeStr=boolean
  Compare To Constant2 : simulink/Logic and Bit Operations/Compare To Constant  relop=>  const=0  OutDataTypeStr=boolean
  Constant : Constant  Value=INS_EXPORT.period  OutDataTypeStr=Inherit: Inherit via back propagation
  Delay : Delay  DelayLength=1
  Detect Rise Positive : simulink/Logic and Bit Operations/Detect Rise Positive  vinit=0  OutDataTypeStr=boolean
  Discrete-Time Integrator : DiscreteIntegrator  IntegratorMethod=Accumulation: Forward Euler  gainval=1  ExternalReset=level  SampleTime=-1  LimitOutput=on  UpperSaturationLimit=1e6  LowerSaturationLimit=0  ICPrevOutput=DiscIntNeverNeededParam  ICPrevScaledInput=DiscIntNeverNeededParam
  Logical Operator : Logic  Operator=NOT  AllPortsSameDT=off  OutDataTypeStr=boolean
  Logical Operator1 : Logic  Operator=OR  AllPortsSameDT=off  OutDataTypeStr=boolean
  Multiply : Product
  y : Outport
  wires:
  Delay/1 -> Logical Operator1/2
  Multiply/1 -> y/1
  Logical Operator1/1 -> Multiply/2, Delay/1
  Detect Rise Positive/1 -> Logical Operator1/1
  Compare To Constant2/1 -> Detect Rise Positive/1
  u/1 -> Compare To Constant1/1, Compare To Constant2/1
  Compare To Constant1/1 -> Discrete-Time Integrator/2
  Constant/1 -> Discrete-Time Integrator/1
  Compare To Constant/1 -> Logical Operator/1
  Logical Operator/1 -> Multiply/1
  Discrete-Time Integrator/1 -> Compare To Constant/1

== system INS/Data_Fusion/Translation_Filter/TF_Data_PreProcess/Transfer_Filter_Control/Sensor_Valid/Vertical_Sensor_Valid/valid_hold ==
  u : Inport
  Compare To Constant : simulink/Logic and Bit Operations/Compare To Constant  relop=>=  const=time_out  OutDataTypeStr=boolean
  Compare To Constant1 : simulink/Logic and Bit Operations/Compare To Constant  relop=>  const=0  OutDataTypeStr=boolean
  Compare To Constant2 : simulink/Logic and Bit Operations/Compare To Constant  relop=>  const=0  OutDataTypeStr=boolean
  Constant : Constant  Value=INS_EXPORT.period  OutDataTypeStr=Inherit: Inherit via back propagation
  Delay : Delay  DelayLength=1
  Detect Rise Positive : simulink/Logic and Bit Operations/Detect Rise Positive  vinit=0  OutDataTypeStr=boolean
  Discrete-Time Integrator : DiscreteIntegrator  IntegratorMethod=Accumulation: Forward Euler  gainval=1  ExternalReset=level  SampleTime=-1  LimitOutput=on  UpperSaturationLimit=1e6  LowerSaturationLimit=0  ICPrevOutput=DiscIntNeverNeededParam  ICPrevScaledInput=DiscIntNeverNeededParam
  Logical Operator : Logic  Operator=NOT  AllPortsSameDT=off  OutDataTypeStr=boolean
  Logical Operator1 : Logic  Operator=OR  AllPortsSameDT=off  OutDataTypeStr=boolean
  Multiply : Product
  y : Outport
  wires:
  Multiply/1 -> y/1
  Logical Operator1/1 -> Multiply/2, Delay/1
  Detect Rise Positive/1 -> Logical Operator1/1
  Compare To Constant2/1 -> Detect Rise Positive/1
  u/1 -> Compare To Constant1/1, Compare To Constant2/1
  Compare To Constant1/1 -> Discrete-Time Integrator/2
  Constant/1 -> Discrete-Time Integrator/1
  Compare To Constant/1 -> Logical Operator/1
  Logical Operator/1 -> Multiply/1
  Discrete-Time Integrator/1 -> Compare To Constant/1
  Delay/1 -> Logical Operator1/2

== system INS/Data_Fusion/Translation_Filter/TF_Data_PreProcess/Transfer_Filter_Control/Sensor_Valid/Vertical_Sensor_Valid/valid_hold1 ==
  u : Inport
  Compare To Constant : simulink/Logic and Bit Operations/Compare To Constant  relop=>=  const=time_out  OutDataTypeStr=boolean
  Compare To Constant1 : simulink/Logic and Bit Operations/Compare To Constant  relop=>  const=0  OutDataTypeStr=boolean
  Compare To Constant2 : simulink/Logic and Bit Operations/Compare To Constant  relop=>  const=0  OutDataTypeStr=boolean
  Constant : Constant  Value=INS_EXPORT.period  OutDataTypeStr=Inherit: Inherit via back propagation
  Delay : Delay  DelayLength=1
  Detect Rise Positive : simulink/Logic and Bit Operations/Detect Rise Positive  vinit=0  OutDataTypeStr=boolean
  Discrete-Time Integrator : DiscreteIntegrator  IntegratorMethod=Accumulation: Forward Euler  gainval=1  ExternalReset=level  SampleTime=-1  LimitOutput=on  UpperSaturationLimit=1e6  LowerSaturationLimit=0  ICPrevOutput=DiscIntNeverNeededParam  ICPrevScaledInput=DiscIntNeverNeededParam
  Logical Operator : Logic  Operator=NOT  AllPortsSameDT=off  OutDataTypeStr=boolean
  Logical Operator1 : Logic  Operator=OR  AllPortsSameDT=off  OutDataTypeStr=boolean
  Multiply : Product
  y : Outport
  wires:
  Discrete-Time Integrator/1 -> Compare To Constant/1
  Logical Operator/1 -> Multiply/1
  Compare To Constant/1 -> Logical Operator/1
  Constant/1 -> Discrete-Time Integrator/1
  Compare To Constant1/1 -> Discrete-Time Integrator/2
  u/1 -> Compare To Constant2/1, Compare To Constant1/1
  Compare To Constant2/1 -> Detect Rise Positive/1
  Detect Rise Positive/1 -> Logical Operator1/1
  Logical Operator1/1 -> Delay/1, Multiply/2
  Multiply/1 -> y/1
  Delay/1 -> Logical Operator1/2

== system INS/Data_Fusion/Translation_Filter/TF_Data_PreProcess/Transfer_Filter_Control/Sensor_Valid/Vertical_Sensor_Valid/valid_hold2 ==
  u : Inport
  Compare To Constant : simulink/Logic and Bit Operations/Compare To Constant  relop=>=  const=time_out  OutDataTypeStr=boolean
  Compare To Constant1 : simulink/Logic and Bit Operations/Compare To Constant  relop=>  const=0  OutDataTypeStr=boolean
  Compare To Constant2 : simulink/Logic and Bit Operations/Compare To Constant  relop=>  const=0  OutDataTypeStr=boolean
  Constant : Constant  Value=INS_EXPORT.period  OutDataTypeStr=Inherit: Inherit via back propagation
  Delay : Delay  DelayLength=1
  Detect Rise Positive : simulink/Logic and Bit Operations/Detect Rise Positive  vinit=0  OutDataTypeStr=boolean
  Discrete-Time Integrator : DiscreteIntegrator  IntegratorMethod=Accumulation: Forward Euler  gainval=1  ExternalReset=level  SampleTime=-1  LimitOutput=on  UpperSaturationLimit=1e6  LowerSaturationLimit=0  ICPrevOutput=DiscIntNeverNeededParam  ICPrevScaledInput=DiscIntNeverNeededParam
  Logical Operator : Logic  Operator=NOT  AllPortsSameDT=off  OutDataTypeStr=boolean
  Logical Operator1 : Logic  Operator=OR  AllPortsSameDT=off  OutDataTypeStr=boolean
  Multiply : Product
  y : Outport
  wires:
  Delay/1 -> Logical Operator1/2
  Multiply/1 -> y/1
  Logical Operator1/1 -> Multiply/2, Delay/1
  Detect Rise Positive/1 -> Logical Operator1/1
  Compare To Constant2/1 -> Detect Rise Positive/1
  u/1 -> Compare To Constant1/1, Compare To Constant2/1
  Compare To Constant1/1 -> Discrete-Time Integrator/2
  Constant/1 -> Discrete-Time Integrator/1
  Compare To Constant/1 -> Logical Operator/1
  Logical Operator/1 -> Multiply/1
  Discrete-Time Integrator/1 -> Compare To Constant/1
